simulink model "generic_src"  (Simulink 10.3)
settings: Solver=ode45  StartTime=0.0  StopTime=inf  RelTol=1e-3  EnableMultiTasking=on
undefined symbols (not defined in the file or in its folder): Area_Front, Area_Rear, ay_max_off, ay_max_on, ay_per_mu_max_off, ay_per_mu_max_on, Brake_ratio, brake_valve_ctrl_kP, cat1mode1_higher, cat1mode1_lower, cat1mode2_higher, cat1mode2_lower, cat1mode3_higher, cat1mode3_lower, cat2mode1_higher, cat2mode1_lower, cat2mode2_higher, cat2mode2_lower, cat2mode3_higher, cat2mode3_lower, delta_vel, diff_lock_fac, diff_lock_off, diff_lock_on, ESP_ctrl_kD, ESP_ctrl_kI, ESP_ctrl_kP, ESP_ctrl_restore_kI, ESP_min_throttle_fac, f_ax, f_slip, g, higherlimit_highvel, higherlimit_lowvel, highervel_fac, highervelocity_fac, InitialConditionForIntegrator, limit_acc, limit_selectlow, limit_starting, limit_vdiff, locktime_throttle, lowerlimit_highvel, lowerlimit_lowvel, lowervel_fac, lowervelocity_fac, min_throttle, MPS2KMPH, MSR_ctrl_kD, MSR_ctrl_kI, MSR_ctrl_kP, MSR_min_throttle_fac, PID_kP_sideslip, PID_kP_yawrate, RADpS2RpM, rBrake, RpM2RADpS, SH_SL_switch, sideslip_vel_corr, sidesplip_deviation_max ... (+35)
libraries: CarMaker4SL x136, simulink x55, simulink_extras x6
(part 9 of 9)

== system generic_src/CarMaker/IPG Vehicle/Brake/HydBrakeCU Example/ESP Controller/ESP General System/ASR/BMR ECU/BMR Controller/Pulsing1 ==
  Constant1 : Constant  Value=1/t_Sensor
  Integrator : Integrator  ExternalReset=either
  Pulse Generator : DiscretePulseGenerator  PulseType=Time based  Period=t_Sensor*2  PulseWidth=50
  SZ : Outport  VectorParamsAs1DForOutWhenUnconnected=off
  wires:
  Integrator/1 -> SZ/1
  Constant1/1 -> Integrator/1
  Pulse Generator/1 -> Integrator/2

== system generic_src/CarMaker/IPG Vehicle/Brake/HydBrakeCU Example/ESP Controller/ESP General System/ASR/BMR ECU/BMR Controller/Signal Mapping ==
  User_In : Inport
  Valve_In_DrivenL : Inport  Port=2
  Valve_Out_DrivenL : Inport  Port=3
  Valve_In_DrivenR : Inport  Port=4
  Valve_Out_DrivenR : Inport  Port=5
  Valve_In_Undriven : Inport  Port=6
  Valve_Out_Undriven : Inport  Port=7
  Valves_Drivenaxle : Inport  Port=8
  Valves_Undrivenaxle : Inport  Port=9
  Bus Selector2 : BusSelector  OutputSignals=User_Drive
  Demux2 : Demux  Outputs=13
  Mux1 : Mux  Inputs=13
  Mux2 : Mux  Inputs=13
  Mux3 : Mux  Inputs=13
  Switch2 : Switch  Criteria=u2 > Threshold  Threshold=1.5
  Switch3 : Switch  Criteria=u2 > Threshold  Threshold=2.5
  Brake Valve_In_FL : Outport  VectorParamsAs1DForOutWhenUnconnected=off
  Brake Valve_In_FR : Outport  Port=2  VectorParamsAs1DForOutWhenUnconnected=off
  Brake Valve_In_RL : Outport  Port=3  VectorParamsAs1DForOutWhenUnconnected=off
  Brake Valve_In_RR : Outport  Port=4  VectorParamsAs1DForOutWhenUnconnected=off
  Brake Valve_Out_FL : Outport  Port=5  VectorParamsAs1DForOutWhenUnconnected=off
  Brake Valve_Out_FR : Outport  Port=6  VectorParamsAs1DForOutWhenUnconnected=off
  Brake Valve_Out_RL : Outport  Port=7  VectorParamsAs1DForOutWhenUnconnected=off
  Brake Valve_Out_RR : Outport  Port=8  VectorParamsAs1DForOutWhenUnconnected=off
  Valve_PV_0 : Outport  Port=9  VectorParamsAs1DForOutWhenUnconnected=off
  Valve_PV_1 : Outport  Port=10  VectorParamsAs1DForOutWhenUnconnected=off
  Valve_SV_0 : Outport  Port=11  VectorParamsAs1DForOutWhenUnconnected=off
  Valve_SV_1 : Outport  Port=12  VectorParamsAs1DForOutWhenUnconnected=off
  Pump Ctrl : Outport  Port=13  VectorParamsAs1DForOutWhenUnconnected=off
  wires:
  Valve_In_Undriven/1 -> Mux2/1, Mux2/2, Mux1/5, Mux1/6
  Valve_Out_Undriven/1 -> Mux2/3, Mux2/4, Mux1/7, Mux1/8
  Valve_In_DrivenR/1 -> Mux2/7, Mux1/3, Mux3/7, Mux3/3
  Valve_In_DrivenL/1 -> Mux3/5, Mux3/1, Mux2/5, Mux1/1
  Valves_Undrivenaxle/1 -> Mux1/12, Mux1/11, Mux2/9, Mux2/10
  Valves_Drivenaxle/1 -> Mux1/9, Mux2/11, Mux2/12, Mux2/13, Mux1/10, Mux1/13, Mux3/10, Mux3/9, Mux3/11, Mux3/12, Mux3/13
  Valve_Out_DrivenL/1 -> Mux3/6, Mux3/2, Mux1/2, Mux2/6
  Valve_Out_DrivenR/1 -> Mux2/8, Mux3/4, Mux3/8, Mux1/4
  User_In/1 -> Bus Selector2/1
  Bus Selector2/1 -> Switch2/2, Switch3/2  "<User_Drive>"
  Switch2/1 -> Switch3/3
  Switch3/1 -> Demux2/1
  Mux1/1 -> Switch2/3
  Mux2/1 -> Switch2/1
  Demux2/1 -> Brake Valve_In_FL/1
  Demux2/2 -> Brake Valve_Out_FL/1
  Demux2/3 -> Brake Valve_In_FR/1
  Demux2/4 -> Brake Valve_Out_FR/1
  Demux2/5 -> Brake Valve_In_RL/1
  Demux2/6 -> Brake Valve_In_RR/1
  Demux2/7 -> Brake Valve_Out_RL/1
  Demux2/8 -> Brake Valve_Out_RR/1
  Demux2/9 -> Valve_PV_0/1
  Demux2/10 -> Valve_SV_0/1
  Demux2/11 -> Valve_PV_1/1
  Demux2/12 -> Valve_SV_1/1
  Demux2/13 -> Pump Ctrl/1
  Mux3/1 -> Switch3/1

== system generic_src/CarMaker/IPG Vehicle/Brake/HydBrakeCU Example/ESP Controller/ESP General System/ASR/BMR ECU/BMR logic/If Action Subsystem6 ==
  Action Port : ActionPort
  Constant : Constant  Value=higherlimit_lowvel
  Constant1 : Constant  Value=lowerlimit_lowvel
  Mux1 : Mux  Inputs=2
  1 : Outport  InitialOutput=[higherlimit_lowvel, lowerlimit_lowvel]  VectorParamsAs1DForOutWhenUnconnected=off
  wires:
  Mux1/1 -> 1/1
  Constant1/1 -> Mux1/2
  Constant/1 -> Mux1/1

== system generic_src/CarMaker/IPG Vehicle/Brake/HydBrakeCU Example/ESP Controller/ESP General System/ASR/BMR ECU/BMR logic/If Action Subsystem7 ==
  Action Port : ActionPort
  Constant : Constant  Value=higherlimit_highvel
  Constant1 : Constant  Value=lowerlimit_highvel
  Mux1 : Mux  Inputs=2
  2 : Outport  InitialOutput=[higherlimit_highvel, lowerlimit_highvel]  VectorParamsAs1DForOutWhenUnconnected=off
  wires:
  Constant/1 -> Mux1/1
  Constant1/1 -> Mux1/2
  Mux1/1 -> 2/1

== system generic_src/CarMaker/IPG Vehicle/Brake/HydBrakeCU Example/ESP Controller/ESP General System/ASR/BMR ECU/BMR logic/operating category ==
  note: Criteria of operating categories (Betriebsarten): Burckhardt: Fahrwerktechnik p.186f.
  v_RL : Inport
  v_RR : Inport  Port=2
  " " : RelationalOperator  Operator=>  OutDataTypeStr=boolean  RndMeth=Nearest
  "  " : Gain  Gain=0.5
  " 1" : RelationalOperator  Operator=<=  OutDataTypeStr=boolean  RndMeth=Nearest
  Add : Sum
  Add1 : Sum
  Constant1 : Constant  Value=delta_vel
  Constant2 : Constant  Value=delta_vel
  Data Type Conversion : DataTypeConversion
  Data Type Conversion1 : DataTypeConversion
  Data Type Conversion2 : DataTypeConversion
  vquer_HA2 : Gain
  vquer_HA3 : Gain  Gain=2
  operating category : Outport  VectorParamsAs1DForOutWhenUnconnected=off
  wires:
  " 1"/1 -> Data Type Conversion1/1
  " "/1 -> Data Type Conversion2/1
  Data Type Conversion/1 -> operating category/1
  Add1/1 -> Data Type Conversion/1
  vquer_HA3/1 -> Add1/2
  vquer_HA2/1 -> Add1/1
  "  "/1 -> " 1"/1, " "/1
  v_RL/1 -> Add/1
  Add/1 -> "  "/1
  v_RR/1 -> Add/2
  Constant2/1 -> " "/2
  Constant1/1 -> " 1"/2
  Data Type Conversion1/1 -> vquer_HA2/1
  Data Type Conversion2/1 -> vquer_HA3/1

== system generic_src/CarMaker/IPG Vehicle/Brake/HydBrakeCU Example/ESP Controller/ESP General System/ASR/MSR ECU/MSR logic/If Action Subsystem ==
  Action Port : ActionPort
  Constant : Constant  Value=cat1mode1_higher
  Constant1 : Constant  Value=cat1mode1_lower
  Mux1 : Mux  Inputs=2
  1.1 : Outport  InitialOutput=[cat1mode1_higher, cat1mode1_lower]  VectorParamsAs1DForOutWhenUnconnected=off
  wires:
  Constant/1 -> Mux1/1
  Constant1/1 -> Mux1/2
  Mux1/1 -> 1.1/1

== system generic_src/CarMaker/IPG Vehicle/Brake/HydBrakeCU Example/ESP Controller/ESP General System/ASR/MSR ECU/MSR logic/If Action Subsystem1 ==
  Action Port : ActionPort
  Constant : Constant  Value=cat1mode2_higher
  Constant1 : Constant  Value=cat1mode2_lower
  Mux1 : Mux  Inputs=2
  1.2 : Outport  InitialOutput=[cat1mode2_higher, cat1mode2_lower]  VectorParamsAs1DForOutWhenUnconnected=off
  wires:
  Mux1/1 -> 1.2/1
  Constant1/1 -> Mux1/2
  Constant/1 -> Mux1/1

== system generic_src/CarMaker/IPG Vehicle/Brake/HydBrakeCU Example/ESP Controller/ESP General System/ASR/MSR ECU/MSR logic/If Action Subsystem2 ==
  Action Port : ActionPort
  Constant2 : Constant  Value=cat1mode3_higher
  Constant3 : Constant  Value=cat1mode3_lower
  Mux1 : Mux  Inputs=2
  1.3 : Outport  InitialOutput=[cat1mode3_higher, cat1mode3_lower]  VectorParamsAs1DForOutWhenUnconnected=off
  wires:
  Mux1/1 -> 1.3/1
  Constant2/1 -> Mux1/1
  Constant3/1 -> Mux1/2

== system generic_src/CarMaker/IPG Vehicle/Brake/HydBrakeCU Example/ESP Controller/ESP General System/ASR/MSR ECU/MSR logic/If Action Subsystem3 ==
  Action Port : ActionPort
  Constant2 : Constant  Value=cat2mode1_higher
  Constant3 : Constant  Value=cat2mode1_lower
  Mux1 : Mux  Inputs=2
  2.1 : Outport  InitialOutput=[cat2mode1_higher, cat2mode1_lower]  VectorParamsAs1DForOutWhenUnconnected=off
  wires:
  Mux1/1 -> 2.1/1
  Constant3/1 -> Mux1/2
  Constant2/1 -> Mux1/1

== system generic_src/CarMaker/IPG Vehicle/Brake/HydBrakeCU Example/ESP Controller/ESP General System/ASR/MSR ECU/MSR logic/If Action Subsystem4 ==
  Action Port : ActionPort
  Constant2 : Constant  Value=cat2mode2_higher
  Constant3 : Constant  Value=cat2mode2_lower
  Mux1 : Mux  Inputs=2
  2.2 : Outport  InitialOutput=[cat2mode2_higher, cat2mode2_lower]  VectorParamsAs1DForOutWhenUnconnected=off
  wires:
  Mux1/1 -> 2.2/1
  Constant2/1 -> Mux1/1
  Constant3/1 -> Mux1/2

== system generic_src/CarMaker/IPG Vehicle/Brake/HydBrakeCU Example/ESP Controller/ESP General System/ASR/MSR ECU/MSR logic/If Action Subsystem5 ==
  Action Port : ActionPort
  Constant2 : Constant  Value=cat2mode3_higher
  Constant3 : Constant  Value=cat2mode3_lower
  Mux1 : Mux  Inputs=2
  2.3 : Outport  InitialOutput=[cat2mode3_higher, cat2mode3_lower]  VectorParamsAs1DForOutWhenUnconnected=off
  wires:
  Mux1/1 -> 2.3/1
  Constant2/1 -> Mux1/1
  Constant3/1 -> Mux1/2

== system generic_src/CarMaker/IPG Vehicle/Brake/HydBrakeCU Example/ESP Controller/ESP General System/ASR/MSR ECU/MSR logic/operating category ==
  note: Criteria of operating categories (Betriebsarten) - Burckhardt: Fahrwerktechnik p.174f.
  v_drivenL : Inport
  v_drivenR : Inport  Port=2
  v_undrivenL : Inport  Port=3
  v_undrivenR : Inport  Port=4
  " " : RelationalOperator  OutDataTypeStr=boolean  RndMeth=Nearest
  " 1" : RelationalOperator  Operator=<=  OutDataTypeStr=boolean  RndMeth=Nearest
  " 2" : RelationalOperator  Operator=>  OutDataTypeStr=boolean  RndMeth=Nearest
  " 3" : RelationalOperator  Operator=<  OutDataTypeStr=boolean  RndMeth=Nearest
  Abs : Abs
  Add : Sum
  Add1 : Sum
  Constant1 : Constant  Value=limit_selectlow
  Constant2 : Constant  Value=SH_SL_switch
  Constant3 : Constant  Value=SH_SL_switch
  Data Type Conversion : DataTypeConversion
  Data Type Conversion1 : DataTypeConversion
  Data Type Conversion2 : DataTypeConversion
  Logical Operator : Logic  AllPortsSameDT=off  OutDataTypeStr=boolean
  Logical Operator1 : Logic  Operator=OR  AllPortsSameDT=off  OutDataTypeStr=boolean
  Subtract : Sum  Inputs=+-
  Subtract1 : Sum  Inputs=+-
  Subtract2 : Sum  Inputs=+-
  vquer_HA : Gain  Gain=0.5
  vquer_HA2 : Gain  Gain=10
  vquer_HA3 : Gain  Gain=20
  category : Outport  VectorParamsAs1DForOutWhenUnconnected=off
  wires:
  v_undrivenR/1 -> Add/2, Subtract1/2
  Add/1 -> vquer_HA/1
  v_undrivenL/1 -> Add/1, Subtract/2
  vquer_HA/1 -> " 2"/1, " 1"/1
  vquer_HA2/1 -> Add1/1
  vquer_HA3/1 -> Add1/2
  Add1/1 -> Data Type Conversion/1
  Data Type Conversion/1 -> category/1
  Logical Operator1/1 -> Data Type Conversion2/1
  " 1"/1 -> Logical Operator/2
  Logical Operator/1 -> Data Type Conversion1/1
  v_drivenL/1 -> Subtract/1
  v_drivenR/1 -> Subtract1/1
  Subtract1/1 -> Subtract2/1
  Subtract/1 -> Subtract2/2
  Subtract2/1 -> Abs/1
  " "/1 -> Logical Operator/1
  " 3"/1 -> Logical Operator1/2
  Abs/1 -> " 3"/1, " "/1
  Constant2/1 -> " "/2
  Constant1/1 -> " 2"/2, " 1"/2
  " 2"/1 -> Logical Operator1/1
  Constant3/1 -> " 3"/2
  Data Type Conversion1/1 -> vquer_HA2/1
  Data Type Conversion2/1 -> vquer_HA3/1

== system generic_src/CarMaker/IPG Vehicle/Brake/HydBrakeCU Example/ESP Controller/ESP General System/ASR/MSR ECU/MSR logic/operating mode ==
  note: Criteria of modes (Arbeitsbereiche) - Burckhardt: Fahrwerktechnik p.174f.
  v_undrivenL : Inport
  v_undrivenR : Inport  Port=2
  " " : RelationalOperator  OutDataTypeStr=boolean  RndMeth=Nearest
  " 1" : RelationalOperator  Operator=<=  OutDataTypeStr=boolean  RndMeth=Nearest
  " 2" : RelationalOperator  Operator=>  OutDataTypeStr=boolean  RndMeth=Nearest
  " 3" : RelationalOperator  Operator=<=  OutDataTypeStr=boolean  RndMeth=Nearest
  AB1 = inaktiv : simulink/Logic and Bit Operations/Compare To Constant  relop=<  const=1  OutDataTypeStr=uint8
  AB1 = inaktiv1 : simulink/Logic and Bit Operations/Compare To Constant  relop=<  const=1  OutDataTypeStr=uint8
  Abs : Abs
  Add : Sum
  Add1 : Sum  Inputs=+++
  Constant1 : Constant  Value=limit_starting
  Constant2 : Constant  Value=limit_acc
  Constant3 : Constant  Value=limit_vdiff
  Constant4 : Constant  Value=MPS2KMPH
  Data Type Conversion{,1..3} (4 alike) : DataTypeConversion
  Derivative : Derivative
  Discrete Filter : DiscreteFilter  Numerator=wheelspeed_filter_num  Denominator=wheelspeed_filter_denom  SampleTime=0.001
  Divide : Product  Inputs=*/
  Logical Operator : Logic  Inputs=3  AllPortsSameDT=off  OutDataTypeStr=boolean
  Logical Operator1 : Logic  AllPortsSameDT=off  OutDataTypeStr=boolean
  Subtract : Sum  Inputs=+-
  v_average_Rear : Gain  Gain=0.5
  vquer_HA2 : Gain
  vquer_HA3 : Gain  Gain=2
  vquer_HA4 : Gain  Gain=3
  mode : Outport  VectorParamsAs1DForOutWhenUnconnected=off
  wires:
  " 1"/1 -> AB1 = inaktiv/1, Data Type Conversion1/1  "mode1 =  active"
  Add/1 -> v_average_Rear/1
  v_undrivenL/1 -> Subtract/1, Add/1
  v_undrivenR/1 -> Add/2, Subtract/2
  v_average_Rear/1 -> " 1"/1, Divide/1, " 2"/1
  Divide/1 -> Discrete Filter/1
  Derivative/1 -> " "/1
  Subtract/1 -> Abs/1
  Abs/1 -> " 3"/1
  Logical Operator/1 -> AB1 = inaktiv1/1, Data Type Conversion2/1
  Logical Operator1/1 -> Data Type Conversion3/1
  AB1 = inaktiv/1 -> Logical Operator1/1
  AB1 = inaktiv1/1 -> Logical Operator1/2
  vquer_HA3/1 -> Add1/2  "mode = 2"
  vquer_HA4/1 -> Add1/3  "mode =3"
  vquer_HA2/1 -> Add1/1  "mode = 1"
  Add1/1 -> Data Type Conversion/1
  " 2"/1 -> Logical Operator/1
  " "/1 -> Logical Operator/2
  Data Type Conversion/1 -> mode/1
  " 3"/1 -> Logical Operator/3
  Discrete Filter/1 -> Derivative/1
  Constant1/1 -> " 2"/2, " 1"/2
  Constant2/1 -> " "/2
  Constant3/1 -> " 3"/2
  Constant4/1 -> Divide/2
  Data Type Conversion1/1 -> vquer_HA2/1
  Data Type Conversion2/1 -> vquer_HA3/1
  Data Type Conversion3/1 -> vquer_HA4/1

== system generic_src/CarMaker/IPG Vehicle/Brake/HydBrakeCU Example/ESP Controller/ESP General System/ASR/MSR ECU/MSR/Gas Controller/Enabled Subsystem ==
  In1 : Inport
  Trigger : TriggerPort  VariantControl=Variant
  Out1 : Outport  VectorParamsAs1DForOutWhenUnconnected=off
  wires:
  In1/1 -> Out1/1

== system generic_src/CarMaker/IPG Vehicle/Brake/HydBrakeCU Example/ESP Controller/ESP General System/ASR/MSR ECU/MSR/Gas Controller/PID Controller ==
  u : Inport
  RESET : Inport  Port=2
  Derivative Gain : Gain  Gain=MSR_ctrl_kD
  Filter : Integrator  ExternalReset=either
  Filter Coefficient : Gain
  Integral Gain : Gain  Gain=MSR_ctrl_kI
  Integrator : Integrator  ExternalReset=either
  Proportional Gain : Gain  Gain=MSR_ctrl_kP
  Sum : Sum  Inputs=+++
  SumD : Sum  Inputs=|+-
  y : Outport  InitialOutput=0  VectorParamsAs1DForOutWhenUnconnected=off
  wires:
  Filter/1 -> SumD/2
  RESET/1 -> Integrator/2, Filter/2
  Sum/1 -> y/1
  Integrator/1 -> Sum/2
  Filter Coefficient/1 -> Filter/1, Sum/3
  Proportional Gain/1 -> Sum/1
  Derivative Gain/1 -> SumD/1
  u/1 -> Integral Gain/1, Derivative Gain/1, Proportional Gain/1
  SumD/1 -> Filter Coefficient/1
  Integral Gain/1 -> Integrator/1

== system generic_src/CarMaker/IPG Vehicle/Brake/HydBrakeCU Example/ESP Controller/ESP General System/ESP/ECU/ECU logic/P Slip angle ==
  x : Inport
  " " : Constant  Value=PID_kP_sideslip
  epsilon11 : Product
  y : Outport  VectorParamsAs1DForOutWhenUnconnected=off
  wires:
  " "/1 -> epsilon11/1
  x/1 -> epsilon11/2
  epsilon11/1 -> y/1

== system generic_src/CarMaker/IPG Vehicle/Brake/HydBrakeCU Example/ESP Controller/ESP General System/ESP/ECU/ECU logic/P Yaw Rate ==
  x : Inport
  " " : Constant  Value=PID_kP_yawrate
  epsilon11 : Product
  y1 : Outport  VectorParamsAs1DForOutWhenUnconnected=off
  wires:
  " "/1 -> epsilon11/1
  x/1 -> epsilon11/2
  epsilon11/1 -> y1/1

== system generic_src/CarMaker/IPG Vehicle/Brake/HydBrakeCU Example/ESP Controller/ESP General System/ESP/ECU/ECU logic/Threshold correction coefficient  as regards vehicle's velocity ==
  v : Inport
  Saturation : Saturate  UpperLimit=1  LowerLimit=0
  Sum2 : Sum  Inputs=+-  InputSameDT=on  SaturateOnIntegerOverflow=on  OutDataTypeStr=Inherit: Same as first input
  b1 : Constant  Value=vel_char_lim_low
  b2 : Constant  Value=vel_char_lim_high
  b3 : Constant  Value=MPS2KMPH
  b4 : Constant  Value=MPS2KMPH
  epsilon1 : Product  Inputs=*/
  epsilon10 : Product  Inputs=/*
  epsilon2 : Product  Inputs=*/
  Threshold correction coefficient : Outport  VectorParamsAs1DForOutWhenUnconnected=off
  wires:
  epsilon10/1 -> Saturation/1
  Sum2/1 -> epsilon10/2
  v/1 -> Sum2/1
  Saturation/1 -> Threshold correction coefficient/1
  epsilon2/1 -> epsilon10/1
  b2/1 -> epsilon2/1
  b3/1 -> epsilon2/2
  b4/1 -> epsilon1/2
  b1/1 -> epsilon1/1
  epsilon1/1 -> Sum2/2

== system generic_src/CarMaker/IPG Vehicle/Brake/HydBrakeCU Example/ESP Controller/ESP General System/ESP/ECU/ECU logic/shut down ESP if v<v lim ==
  note: Transfer Fcn:
      | It enables the ESC to shut down smoothly
      | when the vehicle's velocity becomes lower than v lim
  v : Inport
  v lim ESP : Inport  Port=2
  Data Type Conversion1 : DataTypeConversion
  Gain2 : Gain  OutDataTypeStr=Inherit: Same as input
  Relational Operator : RelationalOperator  OutDataTypeStr=boolean  RndMeth=Nearest
  Transfer Fcn : TransferFcn  Denominator=[0.1 1]
  ON/OFF velocity condition : Outport  VectorParamsAs1DForOutWhenUnconnected=off
  wires:
  v/1 -> Relational Operator/1
  Transfer Fcn/1 -> ON/OFF velocity condition/1
  Relational Operator/1 -> Gain2/1
  v lim ESP/1 -> Relational Operator/2
  Gain2/1 -> Data Type Conversion1/1
  Data Type Conversion1/1 -> Transfer Fcn/1

== system generic_src/CarMaker/IPG Vehicle/Brake/HydBrakeCU Example/ESP Controller/ESP General System/ESP/ECU/Instability detectors/avoids 0 ==
  note: This value has to be low enought
      | to enable the turning radius "r" to
      | be sufficiently large, in order to avoid
      | problems when the steer angle is close to zero
      | (and that the turning radius should be infinty)
  In1 : Inport
  Compare To Zero : simulink/Logic and Bit Operations/Compare To Zero  relop=~=  OutDataTypeStr=uint8
  Constant : Constant  Value=0.00001
  Dead Zone : DeadZone  LowerValue=-0.00001  UpperValue=0.00001  SaturateOnIntegerOverflow=on
  ON/OFF : Relay  OnSwitchValue=0  OffSwitchValue=0  OffOutputValue=-1  ZeroCross=off
  Product7 : Product  RndMeth=Zero
  Switch : Switch  Criteria=u2 > Threshold
  Out1 : Outport  VectorParamsAs1DForOutWhenUnconnected=off
  wires:
  Compare To Zero/1 -> Switch/2
  Dead Zone/1 -> Compare To Zero/1, Switch/1
  Switch/1 -> Out1/1
  In1/1 -> Dead Zone/1, ON/OFF/1
  Product7/1 -> Switch/3
  Constant/1 -> Product7/2
  ON/OFF/1 -> Product7/1

== system generic_src/CarMaker/IPG Vehicle/Brake/HydBrakeCU Example/ESP Controller/ESP General System/ESP/ECU/Instability detectors/avoids 0 again ==
  note: This value has to be lower than "v lim"
      | which is used in the block "response model"
      | to desable the ESP
  In1 : Inport
  Relational Operator : RelationalOperator  OutDataTypeStr=boolean  RndMeth=Nearest
  Switch : Switch  Criteria=u2 > Threshold
  velocity (in m/s) : Constant  Value=3/3.6
  Out1 : Outport  VectorParamsAs1DForOutWhenUnconnected=off
  wires:
  Relational Operator/1 -> Switch/2
  In1/1 -> Relational Operator/1, Switch/1
  velocity (in m/s)/1 -> Relational Operator/2, Switch/3
  Switch/1 -> Out1/1

== system generic_src/CarMaker/IPG Vehicle/Brake/HydBrakeCU Example/ESP Controller/ESP General System/ESP/ECU/Motor management strategy/PID-Controller ==
  u : Inport
  RESET : Inport  Port=2
  Derivative Gain : Gain  Gain=ESP_ctrl_kD
  Filter : Integrator  ExternalReset=either
  Filter Coefficient : Gain
  Integral Gain : Gain  Gain=ESP_ctrl_kI
  Integrator : Integrator  ExternalReset=either
  Proportional Gain : Gain  Gain=ESP_ctrl_kP
  Sum : Sum  Inputs=+++
  SumD : Sum  Inputs=|+-
  y : Outport  InitialOutput=0  VectorParamsAs1DForOutWhenUnconnected=off
  wires:
  Sum/1 -> y/1
  RESET/1 -> Integrator/2, Filter/2
  Derivative Gain/1 -> SumD/1
  Integrator/1 -> Sum/2
  Filter Coefficient/1 -> Filter/1, Sum/3
  Filter/1 -> SumD/2
  Integral Gain/1 -> Integrator/1
  SumD/1 -> Filter Coefficient/1
  Proportional Gain/1 -> Sum/1
  u/1 -> Integral Gain/1, Derivative Gain/1, Proportional Gain/1

== system generic_src/CarMaker/IPG Vehicle/Brake/HydBrakeCU Example/ESP Controller/ESP General System/ESP/ECU/Motor management strategy/restoration to driver ==
  controller in : Inport
  activation on : Inport  Port=2
  driver in : Inport  Port=3
  I-Controller : Subsystem
  Saturation Dynamic1 : simulink/Discontinuities/Saturation Dynamic  OutMin=[]  OutMax=[]  OutDataTypeStr=Inherit: Same as second input  OutDataType=sfix(16)  OutScaling=2^-10  DoSatur=off
  Subtract1 : Sum  Inputs=+-
  lock_signal for n s : Subsystem
  vquer_VA4 : Gain  Gain=0
  vquer_VA5 : Gain
  Control Gas : Outport  VectorParamsAs1DForOutWhenUnconnected=off
  restoration : Outport  Port=2  VectorParamsAs1DForOutWhenUnconnected=off
  wires:
  lock_signal for n s/1(Start_value_locked) -> I-Controller/2(RESET), restoration/1
  Subtract1/1 -> I-Controller/1(u)
  I-Controller/1(y) -> Saturation Dynamic1/2
  vquer_VA4/1 -> Saturation Dynamic1/3
  vquer_VA5/1 -> Saturation Dynamic1/1
  controller in/1 -> I-Controller/3(I0), Subtract1/2
  driver in/1 -> vquer_VA4/1, vquer_VA5/1, Subtract1/1
  activation on/1 -> lock_signal for n s/1(Start_value)
  Saturation Dynamic1/1 -> Control Gas/1

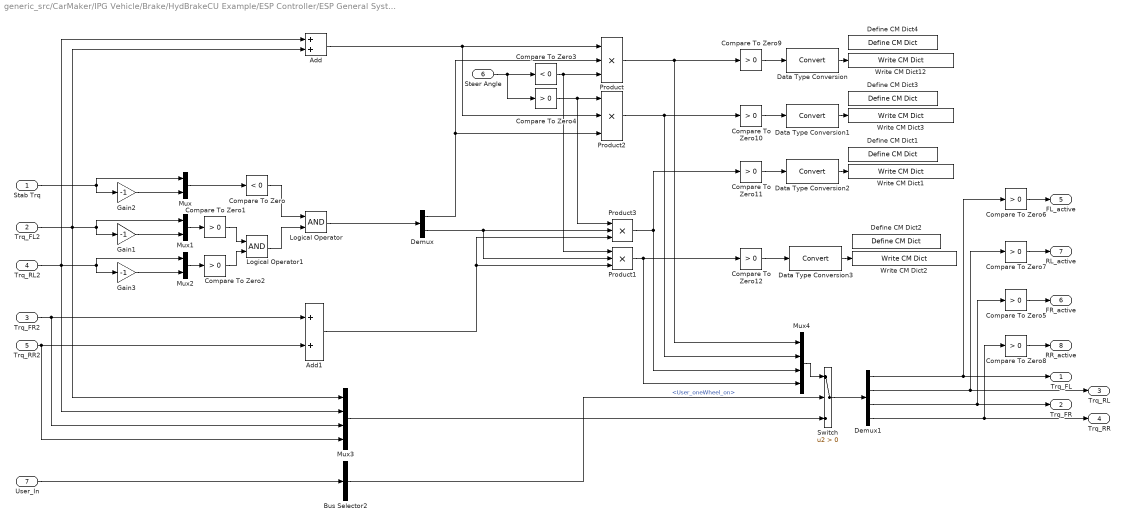
== system generic_src/CarMaker/IPG Vehicle/Brake/HydBrakeCU Example/ESP Controller/ESP General System/ESP/ECU/brake distribution strategy/2Rad ->1Rad ==
  Stab Trq : Inport
  Trq_FL2 : Inport  Port=2
  Trq_FR2 : Inport  Port=3
  Trq_RL2 : Inport  Port=4
  Trq_RR2 : Inport  Port=5
  Steer Angle : Inport  Port=6
  User_In : Inport  Port=7
  Add : Sum
  Add1 : Sum
  Bus Selector2 : BusSelector  OutputSignals=User_oneWheel_on
  Compare To Zero : simulink/Logic and Bit Operations/Compare To Zero  relop=<  OutDataTypeStr=uint8
  Compare To Zero{1..2,4..12} (11 alike) : simulink/Logic and Bit Operations/Compare To Zero  relop=>  OutDataTypeStr=uint8
  Compare To Zero3 : simulink/Logic and Bit Operations/Compare To Zero  relop=<  OutDataTypeStr=uint8
  Data Type Conversion{,1..3} (4 alike) : DataTypeConversion
  Define CM Dict1 : CarMaker4SL/Define CM Dict  xname=ESP.FR_active  xmono=off  xtype=Char  xdvaplace=VC  xnstates=2  xfirststate=0  xinitial=0
  Define CM Dict2 : CarMaker4SL/Define CM Dict  xname=ESP.RR_active  xmono=off  xtype=Char  xdvaplace=VC  xnstates=2  xfirststate=0  xinitial=0
  Define CM Dict3 : CarMaker4SL/Define CM Dict  xname=ESP.RL_active  xmono=off  xtype=Char  xdvaplace=VC  xnstates=2  xfirststate=0  xinitial=0
  Define CM Dict4 : CarMaker4SL/Define CM Dict  xname=ESP.FL_active  xmono=off  xtype=Char  xdvaplace=VC  xnstates=2  xfirststate=0  xinitial=0
  Demux : Demux  Outputs=2
  Demux1 : Demux
  Gain1 : Gain  Gain=-1
  Gain2 : Gain  Gain=-1
  Gain3 : Gain  Gain=-1
  Logical Operator : Logic  AllPortsSameDT=off
  Logical Operator1 : Logic  AllPortsSameDT=off  OutDataTypeStr=boolean
  Mux : Mux  Inputs=2
  Mux1 : Mux  Inputs=2
  Mux2 : Mux  Inputs=2
  Mux3 : Mux
  Mux4 : Mux
  Product{,1..3} (4 alike) : Product  Inputs=3  RndMeth=Zero
  Switch : Switch  Criteria=u2 > Threshold
  Write CM Dict1 : CarMaker4SL/Write CM Dict  xname=ESP.FR_active  xsync=off
  Write CM Dict12 : CarMaker4SL/Write CM Dict  xname=ESP.FL_active  xsync=off
  Write CM Dict2 : CarMaker4SL/Write CM Dict  xname=ESP.RR_active  xsync=off
  Write CM Dict3 : CarMaker4SL/Write CM Dict  xname=ESP.RL_active  xsync=off
  Trq_FL : Outport  VectorParamsAs1DForOutWhenUnconnected=off
  Trq_FR : Outport  Port=2  VectorParamsAs1DForOutWhenUnconnected=off
  Trq_RL : Outport  Port=3  VectorParamsAs1DForOutWhenUnconnected=off
  Trq_RR : Outport  Port=4  VectorParamsAs1DForOutWhenUnconnected=off
  FL_active : Outport  Port=5  VectorParamsAs1DForOutWhenUnconnected=off
  FR_active : Outport  Port=6  VectorParamsAs1DForOutWhenUnconnected=off
  RL_active : Outport  Port=7  VectorParamsAs1DForOutWhenUnconnected=off
  RR_active : Outport  Port=8  VectorParamsAs1DForOutWhenUnconnected=off
  wires:
  Compare To Zero/1 -> Logical Operator/1
  Logical Operator1/1 -> Logical Operator/2
  Logical Operator/1 -> Demux/1
  Compare To Zero1/1 -> Logical Operator1/1
  Compare To Zero2/1 -> Logical Operator1/2
  Stab Trq/1 -> Gain2/1, Mux/1
  Gain2/1 -> Mux/2
  Mux/1 -> Compare To Zero/1
  Trq_FL2/1 -> Gain1/1, Mux1/1, Add/2, Mux3/1
  Gain1/1 -> Mux1/2
  Trq_RL2/1 -> Gain3/1, Mux2/1, Add/1, Mux3/2
  Gain3/1 -> Mux2/2
  Mux2/1 -> Compare To Zero2/1
  Mux1/1 -> Compare To Zero1/1
  Add/1 -> Product/1, Product2/2
  Demux/1 -> Product/2, Product2/3
  Product/1 -> Mux4/1, Compare To Zero9/1
  Add1/1 -> Product3/3, Product1/3
  Demux/2 -> Product3/2, Product1/2
  Product3/1 -> Mux4/3, Compare To Zero11/1
  Trq_FR2/1 -> Add1/1, Mux3/3
  Trq_RR2/1 -> Add1/2, Mux3/4
  Steer Angle/1 -> Compare To Zero3/1, Compare To Zero4/1
  Compare To Zero3/1 -> Product/3, Product1/1
  Product2/1 -> Mux4/2, Compare To Zero10/1
  Compare To Zero4/1 -> Product2/1, Product3/1
  Product1/1 -> Mux4/4, Compare To Zero12/1
  Compare To Zero6/1 -> FL_active/1
  Compare To Zero7/1 -> RL_active/1
  Compare To Zero8/1 -> RR_active/1
  Data Type Conversion/1 -> Write CM Dict12/1
  Mux3/1 -> Switch/3
  Mux4/1 -> Switch/1
  Switch/1 -> Demux1/1
  Demux1/1 -> Trq_FL/1, Compare To Zero6/1
  Demux1/2 -> Trq_RL/1, Compare To Zero7/1
  Demux1/3 -> Trq_FR/1, Compare To Zero5/1
  Demux1/4 -> Trq_RR/1, Compare To Zero8/1
  Bus Selector2/1 -> Switch/2  "<User_oneWheel_on>"
  Compare To Zero9/1 -> Data Type Conversion/1
  Data Type Conversion1/1 -> Write CM Dict3/1
  Compare To Zero10/1 -> Data Type Conversion1/1
  Compare To Zero11/1 -> Data Type Conversion2/1
  Data Type Conversion2/1 -> Write CM Dict1/1
  Data Type Conversion3/1 -> Write CM Dict2/1
  Compare To Zero5/1 -> FR_active/1
  Compare To Zero12/1 -> Data Type Conversion3/1
  User_In/1 -> Bus Selector2/1

== system generic_src/CarMaker/IPG Vehicle/Brake/HydBrakeCU Example/ESP Controller/ESP General System/ESP/helpsignals estimator/mue estimator/estimator_RL ==
  Trq2W_RL : Inport
  Fz_RL : Inport  Port=2
  LongSlip_RL : Inport  Port=3
  Car_vx : Inport  Port=4
  YawRate : Inport  Port=5
  Radius_RL : Inport  Port=6
  " " : simulink/Logic and Bit Operations/Compare To Constant  relop=>=  const=v_min/3.6  OutDataTypeStr=uint8
  "  " : simulink/Logic and Bit Operations/Compare To Constant  relop=>=  const=0.08  OutDataTypeStr=uint8
  "   " : simulink/Logic and Bit Operations/Compare To Constant  relop=<  const=0.2  OutDataTypeStr=uint8
  "    " : simulink/Logic and Bit Operations/Compare To Constant  relop=<=  const=0.15  OutDataTypeStr=uint8
  Abs : Abs
  Compare To Constant2 : simulink/Logic and Bit Operations/Compare To Constant  relop=>  const=-0.05  OutDataTypeStr=uint8
  Compare To Zero : simulink/Logic and Bit Operations/Compare To Zero  relop=>  OutDataTypeStr=uint8
  Compare To Zero1 : simulink/Logic and Bit Operations/Compare To Zero  relop=<  OutDataTypeStr=uint8
  Compare To Zero2 : simulink/Logic and Bit Operations/Compare To Zero  relop=>  OutDataTypeStr=uint8
  Compare To Zero3 : simulink/Logic and Bit Operations/Compare To Zero  relop=>  OutDataTypeStr=uint8
  Constant : Constant  Value=0
  Constant1 : Constant
  Divide1 : Product  Inputs=**
  Divide2 : Product  Inputs=*/
  Divide3 : Product  Inputs=*/
  Gain : Gain  Gain=-1
  Gain1 : Gain  Gain=0.5
  Logical Operator : Logic  Inputs=4  AllPortsSameDT=off  OutDataTypeStr=boolean
  Logical Operator1 : Logic  AllPortsSameDT=off  OutDataTypeStr=boolean
  Logical Operator2 : Logic  AllPortsSameDT=off  OutDataTypeStr=boolean
  Lookup Table : Lookup  InputValues=[0.8 1.8 5.2 6.9 9.5]  Table=[0.1 0.2 0.5 0.7 1]  LookUpMeth=Interpolation-Use End Values
  Memory : Memory
  Subtract : Sum  Inputs=+-
  Subtract1 : Sum
  Switch : Switch  Criteria=u2 > Threshold
  Switch1 : Switch  Criteria=u2 > Threshold
  Triggered Subsystem : Subsystem  TreatAsAtomicUnit=on
  Triggered Subsystem1 : Subsystem  TreatAsAtomicUnit=on
  mue_est_RL : Outport  VectorParamsAs1DForOutWhenUnconnected=off
  wires:
  Divide1/1 -> Divide2/2
  Divide2/1 -> Divide3/1
  "  "/1 -> Logical Operator/1
  "    "/1 -> Logical Operator/2
  Logical Operator/1 -> Switch/2
  Divide3/1 -> Switch/1
  Switch/1 -> Lookup Table/1
  Constant/1 -> Switch/3
  Gain/1 -> Divide3/2, "  "/1, "    "/1
  Lookup Table/1 -> Memory/1, Subtract/1, Triggered Subsystem/1(In1), Triggered Subsystem1/1(In1)
  Memory/1 -> Subtract/2
  Subtract/1 -> Compare To Zero1/1, Compare To Constant2/1, Compare To Zero/1
  Compare To Zero/1 -> Triggered Subsystem/Trigger
  Compare To Zero1/1 -> Logical Operator1/1
  Compare To Constant2/1 -> Logical Operator1/2
  Logical Operator1/1 -> Triggered Subsystem1/Trigger
  Car_vx/1 -> " "/1
  " "/1 -> Logical Operator/3
  Triggered Subsystem/1(Out1) -> Subtract1/1, Compare To Zero2/1
  Triggered Subsystem1/1(Out1) -> Compare To Zero3/1, Subtract1/2
  Compare To Zero2/1 -> Logical Operator2/1
  Compare To Zero3/1 -> Logical Operator2/2
  Logical Operator2/1 -> Switch1/2
  Subtract1/1 -> Gain1/1
  Constant1/1 -> Switch1/3
  Gain1/1 -> Switch1/1
  Trq2W_RL/1 -> Divide2/1
  Fz_RL/1 -> Divide1/1
  Radius_RL/1 -> Divide1/2
  LongSlip_RL/1 -> Gain/1
  Switch1/1 -> mue_est_RL/1
  YawRate/1 -> Abs/1
  Abs/1 -> "   "/1
  "   "/1 -> Logical Operator/4

== system generic_src/CarMaker/IPG Vehicle/Brake/HydBrakeCU Example/ESP Controller/ESP General System/ESP/helpsignals estimator/mue estimator/estimator_RR ==
  Trq2W_RR : Inport
  Fz_RR : Inport  Port=2
  LongSlip_RR : Inport  Port=3
  Car_vx : Inport  Port=4
  YawRate : Inport  Port=5
  Radius_RR : Inport  Port=6
  " " : simulink/Logic and Bit Operations/Compare To Constant  relop=>=  const=v_min/3.6  OutDataTypeStr=uint8
  "  " : simulink/Logic and Bit Operations/Compare To Constant  relop=>=  const=0.08  OutDataTypeStr=uint8
  "   " : simulink/Logic and Bit Operations/Compare To Constant  relop=<  const=0.2  OutDataTypeStr=uint8
  "    " : simulink/Logic and Bit Operations/Compare To Constant  relop=<=  const=0.15  OutDataTypeStr=uint8
  Abs : Abs
  Compare To Constant2 : simulink/Logic and Bit Operations/Compare To Constant  relop=>  const=-0.05  OutDataTypeStr=uint8
  Compare To Zero : simulink/Logic and Bit Operations/Compare To Zero  relop=>  OutDataTypeStr=uint8
  Compare To Zero1 : simulink/Logic and Bit Operations/Compare To Zero  relop=<  OutDataTypeStr=uint8
  Compare To Zero2 : simulink/Logic and Bit Operations/Compare To Zero  relop=>  OutDataTypeStr=uint8
  Compare To Zero3 : simulink/Logic and Bit Operations/Compare To Zero  relop=>  OutDataTypeStr=uint8
  Constant : Constant  Value=0
  Constant1 : Constant
  Divide1 : Product  Inputs=**
  Divide2 : Product  Inputs=*/
  Divide3 : Product  Inputs=*/
  Gain : Gain  Gain=-1
  Gain1 : Gain  Gain=0.5
  Logical Operator : Logic  Inputs=4  AllPortsSameDT=off  OutDataTypeStr=boolean
  Logical Operator1 : Logic  AllPortsSameDT=off  OutDataTypeStr=boolean
  Logical Operator2 : Logic  AllPortsSameDT=off  OutDataTypeStr=boolean
  Lookup Table : Lookup  InputValues=[0.8 1.8 5.2 6.9 9.5]  Table=[0.1 0.2 0.5 0.7 1]  LookUpMeth=Interpolation-Use End Values
  Memory : Memory
  Subtract : Sum  Inputs=+-
  Subtract1 : Sum
  Switch : Switch  Criteria=u2 > Threshold
  Switch1 : Switch  Criteria=u2 > Threshold
  Triggered Subsystem : Subsystem  TreatAsAtomicUnit=on
  Triggered Subsystem1 : Subsystem  TreatAsAtomicUnit=on
  mue_est_RR : Outport  VectorParamsAs1DForOutWhenUnconnected=off
  wires:
  Divide1/1 -> Divide2/2
  Divide2/1 -> Divide3/1
  "  "/1 -> Logical Operator/1
  "    "/1 -> Logical Operator/2
  Logical Operator/1 -> Switch/2
  Divide3/1 -> Switch/1
  Switch/1 -> Lookup Table/1
  Constant/1 -> Switch/3
  Gain/1 -> Divide3/2, "  "/1, "    "/1
  Lookup Table/1 -> Memory/1, Subtract/1, Triggered Subsystem/1(In1), Triggered Subsystem1/1(In1)
  Memory/1 -> Subtract/2
  Subtract/1 -> Compare To Zero1/1, Compare To Constant2/1, Compare To Zero/1
  Compare To Zero/1 -> Triggered Subsystem/Trigger
  Compare To Zero1/1 -> Logical Operator1/1
  Compare To Constant2/1 -> Logical Operator1/2
  Logical Operator1/1 -> Triggered Subsystem1/Trigger
  Car_vx/1 -> " "/1
  " "/1 -> Logical Operator/3
  Triggered Subsystem/1(Out1) -> Subtract1/1, Compare To Zero2/1
  Triggered Subsystem1/1(Out1) -> Compare To Zero3/1, Subtract1/2
  Compare To Zero2/1 -> Logical Operator2/1
  Compare To Zero3/1 -> Logical Operator2/2
  Logical Operator2/1 -> Switch1/2
  Subtract1/1 -> Gain1/1
  Constant1/1 -> Switch1/3
  Gain1/1 -> Switch1/1
  Trq2W_RR/1 -> Divide2/1
  Fz_RR/1 -> Divide1/1
  Radius_RR/1 -> Divide1/2
  LongSlip_RR/1 -> Gain/1
  Switch1/1 -> mue_est_RR/1
  YawRate/1 -> Abs/1
  Abs/1 -> "   "/1
  "   "/1 -> Logical Operator/4

== system generic_src/CarMaker/IPG Vehicle/Brake/HydBrakeCU Example/ESP Controller/ESP General System/ABS/ABS ECU/select_low/ABS_ValveCtrl_rear/Duty ==
  Constant1 : Constant  Value=1/t_Sensor
  Integrator : Integrator  ExternalReset=either
  Pulse Generator : DiscretePulseGenerator  PulseType=Time based  Period=t_Sensor*2  PulseWidth=50
  SZ : Outport  VectorParamsAs1DForOutWhenUnconnected=off
  wires:
  Integrator/1 -> SZ/1
  Pulse Generator/1 -> Integrator/2
  Constant1/1 -> Integrator/1

== system generic_src/CarMaker/IPG Vehicle/Brake/HydBrakeCU Example/ESP Controller/ESP General System/ESP/ECU/Motor management strategy/restoration to driver/I-Controller ==
  u : Inport
  RESET : Inport  Port=2
  I0 : Inport  Port=3
  Integral Gain : Gain  Gain=ESP_ctrl_restore_kI
  Integrator : Integrator  ExternalReset=either  InitialConditionSource=external  InitialCondition=InitialConditionForIntegrator
  y : Outport  InitialOutput=0  VectorParamsAs1DForOutWhenUnconnected=off
  wires:
  Integrator/1 -> y/1
  Integral Gain/1 -> Integrator/1
  RESET/1 -> Integrator/2
  u/1 -> Integral Gain/1
  I0/1 -> Integrator/3

== system generic_src/CarMaker/IPG Vehicle/Brake/HydBrakeCU Example/ESP Controller/ESP General System/ESP/ECU/Motor management strategy/restoration to driver/lock_signal for n s ==
  Start_value : Inport
  " " : simulink/Logic and Bit Operations/Compare To Constant  relop=>  const=0  OutDataTypeStr=uint8
  Constant : Constant  Value=locktime_throttle
  Data Type Conversion : DataTypeConversion
  Integrator : Integrator  ExternalReset=falling
  Logical Operator3 : Logic  AllPortsSameDT=off  OutDataTypeStr=boolean
  Relational Operator : RelationalOperator  Operator=<=  OutDataTypeStr=boolean  RndMeth=Nearest
  Triggered Subsystem : Subsystem  TreatAsAtomicUnit=on
  Start_value_locked : Outport  VectorParamsAs1DForOutWhenUnconnected=off
  wires:
  Start_value/1 -> Triggered Subsystem/Trigger, Integrator/2
  Integrator/1 -> " "/1, Relational Operator/1
  Triggered Subsystem/1(Out1) -> Integrator/1
  " "/1 -> Logical Operator3/1
  Relational Operator/1 -> Logical Operator3/2
  Data Type Conversion/1 -> Start_value_locked/1
  Logical Operator3/1 -> Data Type Conversion/1
  Constant/1 -> Relational Operator/2

== system generic_src/CarMaker/IPG Vehicle/Brake/HydBrakeCU Example/ESP Controller/ESP General System/ESP/helpsignals estimator/mue estimator/estimator_RL/Triggered Subsystem ==
  In1 : Inport
  Trigger : TriggerPort  VariantControl=Variant
  Out1 : Outport  VectorParamsAs1DForOutWhenUnconnected=off
  wires:
  In1/1 -> Out1/1

== system generic_src/CarMaker/IPG Vehicle/Brake/HydBrakeCU Example/ESP Controller/ESP General System/ESP/helpsignals estimator/mue estimator/estimator_RL/Triggered Subsystem1 ==
  In1 : Inport
  Trigger : TriggerPort  VariantControl=Variant
  Out1 : Outport  VectorParamsAs1DForOutWhenUnconnected=off
  wires:
  In1/1 -> Out1/1

== system generic_src/CarMaker/IPG Vehicle/Brake/HydBrakeCU Example/ESP Controller/ESP General System/ESP/helpsignals estimator/mue estimator/estimator_RR/Triggered Subsystem ==
  In1 : Inport
  Trigger : TriggerPort  VariantControl=Variant
  Out1 : Outport  VectorParamsAs1DForOutWhenUnconnected=off
  wires:
  In1/1 -> Out1/1

== system generic_src/CarMaker/IPG Vehicle/Brake/HydBrakeCU Example/ESP Controller/ESP General System/ESP/helpsignals estimator/mue estimator/estimator_RR/Triggered Subsystem1 ==
  In1 : Inport
  Trigger : TriggerPort  VariantControl=Variant
  Out1 : Outport  VectorParamsAs1DForOutWhenUnconnected=off
  wires:
  In1/1 -> Out1/1

== system generic_src/CarMaker/IPG Vehicle/Brake/HydBrakeCU Example/ESP Controller/ESP General System/ESP/ECU/Motor management strategy/restoration to driver/lock_signal for n s/Triggered Subsystem ==
  Trigger : TriggerPort  TriggerType=falling  VariantControl=Variant
  Constant1 : Constant
  Out1 : Outport  InitialOutput=[0]  VectorParamsAs1DForOutWhenUnconnected=off
  wires:
  Constant1/1 -> Out1/1
